simulink model "Energy_storage_blocks"  (R2025b)
settings: Solver=VariableStepAuto  StartTime=0.0  StopTime=1000  RelTol=1e-3
values from neighbouring files (symbols this model uses):
  R = 0.01    [DATA_LI_ION_CELL.mat]
undefined symbols (not defined in the file or in its folder): BATTERY_1, DC_CAPACITIVE_FILTER_1, DC_INDUCTIVE_FILTER_1, DCDC_CONVERTER_1, DCDC_CONVERTER_CONTROLLER_1, F, L
libraries: simulink x2
settings Model: Creator=barra  LastModifiedBy=DNI 76350607

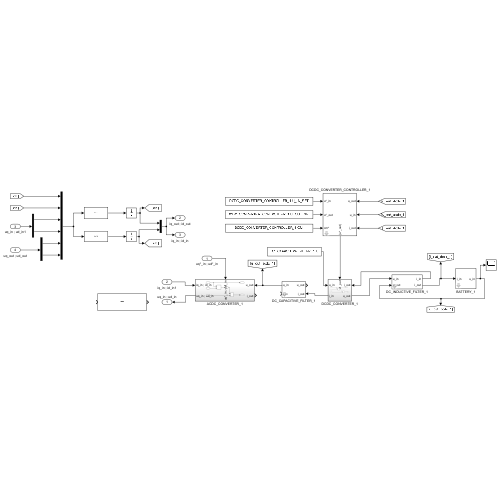
[thumbnail: Simulink's stored preview of the top-level diagram]
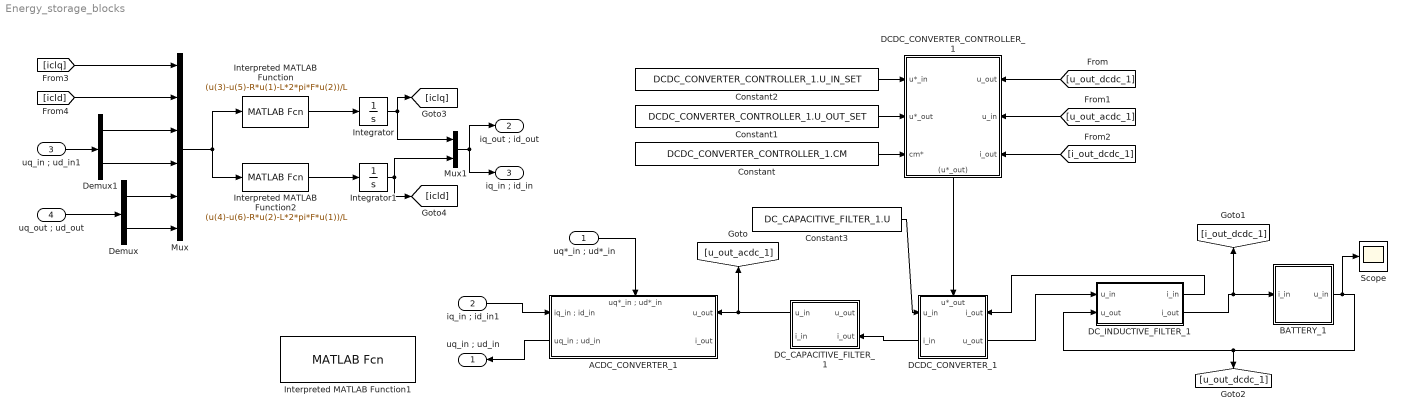
== system Energy_storage_blocks ==
  uq*_in ; ud*_in : Inport
  iq_in ; id_in1 : Inport  Port=2
  uq_in ; ud_in1 : Inport  Port=3
  uq_out ; ud_out : Inport  Port=4
  ACDC_CONVERTER_1 : Subsystem
      settings: PortSchema="{\"entries\":[{\"content\":{\"sides\":[{\"content\":{\"connectorIds\":[\"In1\",\"Out2\"]},\"type\":\"ConnectorPlacement.EquallySpacedRectSide\",\"uuid\":\"8c383f18-b1b8-414a-9022-83b924be4ee1\"},{\"content\":{\"connectorIds\":[\"In3\",\"Out1\"],\"side\":\"RIGHT\"},\"type\":\"ConnectorPlacement.EquallySpacedRectSide\",\"uuid\":\"b6aa94b4-5558-4a55-88af-197c4f32b9d6\"},{\"content\":{\"connectorIds\":[\"In2\"],\"side\":\"TOP\"},\"type\":\"ConnectorPlacement.EquallySpacedRectSide\",\"uuid\":\"f27b2a4b-2b11-4cc8-a3ae-660875af7a27\"}]},\"type\":\"ConnectorPlacement.EquallySpacedConnector\",\"uuid\":\"ed3a75f0-3b30-4418-b841-97d400508208\"}],\"packageUris\":[\"http://schema.mathworks.com/mf0/Connector/R2020b\"],\"version\":\"1.0\"}"
  BATTERY_1 : Subsystem  mask{R=BATTERY_1.R, EFF=BATTERY_1.EFF, C=BATTERY_1.C, OCV_LUT=BATTERY_1.OCV_LUT, SOC_LUT=BATTERY_1.SOC_LUT, SOC_INI=BATTERY_1.SOC_INI}
      mask prompts: R "Internal resistance (Ohm)"; EFF "Efficiency (p.u.)"; C "Capacity (Ah)"; OCV_LUT "Open Circuit Voltage OCV (V)"; SOC_LUT "Open Circuit Voltage SOC (p.u.)"; SOC_INI "Initial SOC (p.u.)"
      mask DialogControl DescTextVar Prompt: Battery.
  Constant : Constant  Value=DCDC_CONVERTER_CONTROLLER_1.CM
  Constant1 : Constant  Value=DCDC_CONVERTER_CONTROLLER_1.U_OUT_SET
  Constant2 : Constant  Value=DCDC_CONVERTER_CONTROLLER_1.U_IN_SET
  Constant3 : Constant  Value=DC_CAPACITIVE_FILTER_1.U
  DCDC_CONVERTER_1 : Subsystem
      settings: PortSchema="{\"entries\":[{\"content\":{\"sides\":[{\"content\":{\"connectorIds\":[\"In1\",\"Out2\"]},\"type\":\"ConnectorPlacement.EquallySpacedRectSide\",\"uuid\":\"16b79129-35bd-40e4-9150-a907a2dc894e\"},{\"content\":{\"connectorIds\":[\"In3\",\"Out1\"],\"side\":\"RIGHT\"},\"type\":\"ConnectorPlacement.EquallySpacedRectSide\",\"uuid\":\"aebd2ac3-6df7-4285-ab4e-40db8a096b32\"},{\"content\":{\"connectorIds\":[\"In2\"],\"side\":\"TOP\"},\"type\":\"ConnectorPlacement.EquallySpacedRectSide\",\"uuid\":\"705a8761-481f-43da-b8bb-0b2cee8f59be\"}]},\"type\":\"ConnectorPlacement.EquallySpacedConnector\",\"uuid\":\"5da3bf74-39a7-4819-a145-9938271c38b8\"}],\"packageUris\":[\"http://schema.mathworks.com/mf0/Connector/R2020b\"],\"version\":\"1.0\"}"
  DCDC_CONVERTER_CONTROLLER_1 : Subsystem  mask{I_MAX=DCDC_CONVERTER_1.I_OUT, U_IN=DCDC_CONVERTER_1.U_IN, KPU=DCDC_CONVERTER_CONTROLLER_1.KPU, KIU=DCDC_CONVERTER_CONTROLLER_1.KIU, KPI=DCDC_CONVERTER_CONTROLLER_1.KPI, KII=DCDC_CONVERTER_CONTROLLER_1.KII, INT_INI=DCDC_CONVERTER_CONTROLLER_1.INT_INI}
      mask prompts: I_MAX "Rated output current, (A)"; U_IN "Rated input voltage, (V)"; KPU "Output voltage controller, Kp (-)"; KIU "Output voltage controller, Ki (-)"; KPI "Output current controller, Kp (-)"; KII "Output current controller, Ki (-)"; INT_INI "Initial condition, current controller"
      settings: PortSchema="{\"entries\":[{\"content\":{\"sides\":[{\"content\":{\"connectorIds\":[\"In1\",\"In2\",\"In3\"]},\"type\":\"ConnectorPlacement.EquallySpacedRectSide\",\"uuid\":\"a907ae50-daf0-48ac-8972-584c22ec23bc\"},{\"content\":{\"connectorIds\":[\"In4\",\"In5\",\"In6\"],\"side\":\"RIGHT\"},\"type\":\"ConnectorPlacement.EquallySpacedRectSide\",\"uuid\":\"c451cec1-46fa-46e7-84b6-32aef918d9a7\"},{\"content\":{\"side\":\"TOP\"},\"type\":\"ConnectorPlacement.EquallySpacedRectSide\",\"uuid\":\"5fac8104-b6a5-4db9-beed-e5f35f7b50c1\"},{\"content\":{\"connectorIds\":[\"Out1\"],\"side\":\"BOTTOM\"},\"type\":\"ConnectorPlacement.EquallySpacedRectSide\",\"uuid\":\"880ffd14-00d8-4352-9ce0-8d5bb61b95c0\"}]},\"type\":\"ConnectorPlacement.EquallySpacedConnector\",\"uuid\":\"6bb2e475-6dd4-45a2-84d8-2ce6e01c7f10\"}],\"packageUris\":[\"http://schema.mathworks.com/mf0/Connector/R2020b\"],\"version\":\"1.0\"}"
      mask DialogControl DescGroupVar Prompt: Bidirectional buck-boost DCDC converter controller.
      mask DialogControl Container2 Prompt: Parameters
  DC_CAPACITIVE_FILTER_1 : Subsystem  mask{C=DC_CAPACITIVE_FILTER_1.C, U=DC_CAPACITIVE_FILTER_1.U}
      mask prompts: C "Capacitance (F)"; U "Initial voltage (V)"
      settings: PortSchema="{\"entries\":[{\"content\":{\"sides\":[{\"content\":{\"connectorIds\":[\"Out2\",\"In1\"]},\"type\":\"ConnectorPlacement.EquallySpacedRectSide\",\"uuid\":\"bcba4002-f43e-4ceb-8615-0b17579625fa\"},{\"content\":{\"connectorIds\":[\"Out1\",\"In2\"],\"side\":\"RIGHT\"},\"type\":\"ConnectorPlacement.EquallySpacedRectSide\",\"uuid\":\"6d888d39-6fd7-425a-a11e-fe4702aa9d62\"},{\"content\":{\"side\":\"TOP\"},\"type\":\"ConnectorPlacement.EquallySpacedRectSide\",\"uuid\":\"f7aa08bb-58ae-4915-b02f-c1bef0b1235c\"}]},\"type\":\"ConnectorPlacement.EquallySpacedConnector\",\"uuid\":\"fb6703e1-98b4-4d7d-a745-8e02b5eae5ed\"}],\"packageUris\":[\"http://schema.mathworks.com/mf0/Connector/R2020b\"],\"version\":\"1.0\"}"
      mask DialogControl DescGroupVar Prompt: DC capacitive filter
  DC_INDUCTIVE_FILTER_1 : Subsystem  mask{L=DC_INDUCTIVE_FILTER_1.L}
      mask prompts: L "Inductance (H)"
      mask DialogControl DescGroupVar Prompt: DC inductive filter
  Demux : Demux  Outputs=2
  Demux1 : Demux  Outputs=2
  Integrator : Integrator
  Integrator1 : Integrator
  Interpreted MATLAB Function : MATLABFcn  MATLABFcn=(u(3)-u(5)-R*u(1)-L*2*pi*F*u(2))/L  OutputDimensions=1
  Interpreted MATLAB Function1 : MATLABFcn
  Interpreted MATLAB Function2 : MATLABFcn  MATLABFcn=(u(4)-u(6)-R*u(2)-L*2*pi*F*u(1))/L  OutputDimensions=1
  Mux : Mux  Inputs=6
  Mux1 : Mux  Inputs=2
  Scope : Scope
      settings: ActiveDisplayYMinimum=577.2389529667704  ActiveDisplayYMaximum=641.19342329906692
  uq_in ; ud_in : Outport
  iq_out ; id_out : Outport  Port=2
  iq_in ; id_in : Outport  Port=3
  wires:
  BATTERY_1/1(u_in) -> Scope/1, DC_INDUCTIVE_FILTER_1/2(u_out), [u_out_dcdc_1]
  DC_INDUCTIVE_FILTER_1/2(i_out) -> [i_out_dcdc_1], BATTERY_1/1(i_in)
  DC_INDUCTIVE_FILTER_1/1(i_in) -> DCDC_CONVERTER_1/3(i_out)
  DCDC_CONVERTER_1/1(u_out) -> DC_INDUCTIVE_FILTER_1/1(u_in)
  DCDC_CONVERTER_1/2(i_in) -> DC_CAPACITIVE_FILTER_1/2(i_out)
  iq_in ; id_in1/1 -> ACDC_CONVERTER_1/1(iq_in ; id_in)
  ACDC_CONVERTER_1/2(uq_in ; ud_in) -> uq_in ; ud_in/1
  uq*_in ; ud*_in/1 -> ACDC_CONVERTER_1/2(uq*_in ; ud*_in)
  DCDC_CONVERTER_CONTROLLER_1/1((u*_out)) -> DCDC_CONVERTER_1/2(u*_out)
  [i_out_dcdc_1] -> DCDC_CONVERTER_CONTROLLER_1/6(i_out)
  [u_out_dcdc_1] -> DCDC_CONVERTER_CONTROLLER_1/4(u_out)
  Constant2/1 -> DCDC_CONVERTER_CONTROLLER_1/1(u*_in)
  Constant1/1 -> DCDC_CONVERTER_CONTROLLER_1/2(u*_out)
  Constant/1 -> DCDC_CONVERTER_CONTROLLER_1/3(cm*)
  DC_CAPACITIVE_FILTER_1/2(u_in) -> [u_out_acdc_1], ACDC_CONVERTER_1/3(u_out)
  Constant3/1 -> DCDC_CONVERTER_1/1(u_in)
  [u_out_acdc_1] -> DCDC_CONVERTER_CONTROLLER_1/5(u_in)
  Demux/2 -> Mux/6
  Demux/1 -> Mux/5
  Demux1/1 -> Mux/3
  Demux1/2 -> Mux/4
  uq_in ; ud_in1/1 -> Demux1/1
  uq_out ; ud_out/1 -> Demux/1
  Mux/1 -> Interpreted MATLAB Function/1, Interpreted MATLAB Function2/1
  Interpreted MATLAB Function/1 -> Integrator/1
  Interpreted MATLAB Function2/1 -> Integrator1/1
  Integrator1/1 -> [icld], Mux1/2
  Integrator/1 -> [iclq], Mux1/1
  Mux1/1 -> iq_in ; id_in/1, iq_out ; id_out/1
  [iclq] -> Mux/1
  [icld] -> Mux/2

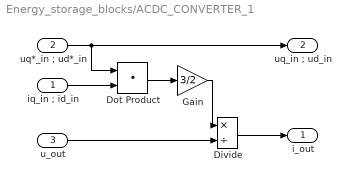
== system Energy_storage_blocks/ACDC_CONVERTER_1 ==
  iq_in ; id_in : Inport
  uq*_in ; ud*_in : Inport  Port=2
  u_out : Inport  Port=3
  Divide : Product  Inputs=*/
  Dot Product : DotProduct  OutDataTypeStr=Inherit: Inherit via internal rule
  Gain : Gain  Gain=3/2
  i_out : Outport
  uq_in ; ud_in : Outport  Port=2
  wires:
  Dot Product/1 -> Gain/1
  Gain/1 -> Divide/1
  uq*_in ; ud*_in/1 -> uq_in ; ud_in/1, Dot Product/1
  Divide/1 -> i_out/1
  u_out/1 -> Divide/2
  iq_in ; id_in/1 -> Dot Product/2

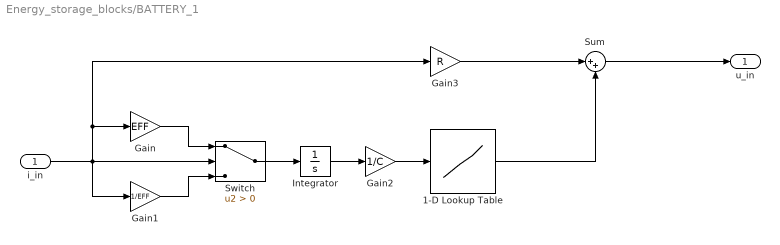
== system Energy_storage_blocks/BATTERY_1 ==
  i_in : Inport
  1-D Lookup Table : Lookup_n-D  NumberOfTableDimensions=1  BreakpointsForDimension1=SOC_LUT  Table=OCV_LUT  InternalRulePriority=Speed  RndMeth=Simplest
  Gain : Gain  Gain=EFF
  Gain1 : Gain  Gain=1/EFF
  Gain2 : Gain  Gain=1/C
  Gain3 : Gain  Gain=R
  Integrator : Integrator  InitialCondition=SOC_INI*C
  Sum : Sum  Inputs=|++
  Switch : Switch  Criteria=u2 > Threshold  SaturateOnIntegerOverflow=off  InputSameDT=off
  u_in : Outport
  wires:
  i_in/1 -> Gain1/1, Gain3/1, Gain/1, Switch/2
  Sum/1 -> u_in/1
  Gain2/1 -> 1-D Lookup Table/1
  Gain1/1 -> Switch/3
  Gain/1 -> Switch/1
  1-D Lookup Table/1 -> Sum/2
  Switch/1 -> Integrator/1
  Gain3/1 -> Sum/1
  Integrator/1 -> Gain2/1

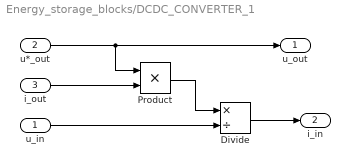
== system Energy_storage_blocks/DCDC_CONVERTER_1 ==
  u_in : Inport
  u*_out : Inport  Port=2
  i_out : Inport  Port=3
  Divide : Product  Inputs=*/
  Product : Product
  u_out : Outport
  i_in : Outport  Port=2
  wires:
  Divide/1 -> i_in/1
  Product/1 -> Divide/1
  u_in/1 -> Divide/2
  u*_out/1 -> u_out/1, Product/1
  i_out/1 -> Product/2

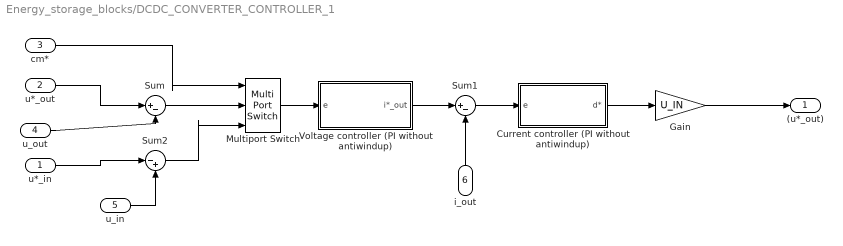
== system Energy_storage_blocks/DCDC_CONVERTER_CONTROLLER_1 ==
  u*_in : Inport
  u*_out : Inport  Port=2
  cm* : Inport  Port=3
  u_out : Inport  Port=4
  u_in : Inport  Port=5
  i_out : Inport  Port=6
  Current controller (PI without antiwindup) : Subsystem
  Gain : Gain  Gain=U_IN
  Multiport Switch : MultiPortSwitch  Inputs=2  SaturateOnIntegerOverflow=off  InputSameDT=off
  Sum : Sum  Inputs=|+-
  Sum1 : Sum  Inputs=|+-
  Sum2 : Sum  Inputs=|-+
  Voltage controller (PI without antiwindup) : Subsystem
  (u*_out) : Outport
  wires:
  Current controller (PI without antiwindup)/1(d*) -> Gain/1
  Sum/1 -> Multiport Switch/2
  i_out/1 -> Sum1/2
  Voltage controller (PI without antiwindup)/1(i*_out) -> Sum1/1
  cm*/1 -> Multiport Switch/1
  Gain/1 -> (u*_out)/1
  u_in/1 -> Sum2/2
  Sum1/1 -> Current controller (PI without antiwindup)/1(e)
  u*_out/1 -> Sum/1
  u*_in/1 -> Sum2/1
  u_out/1 -> Sum/2
  Multiport Switch/1 -> Voltage controller (PI without antiwindup)/1(e)
  Sum2/1 -> Multiport Switch/3

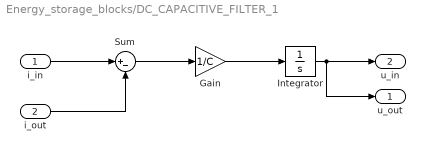
== system Energy_storage_blocks/DC_CAPACITIVE_FILTER_1 ==
  i_in : Inport
  i_out : Inport  Port=2
  Gain : Gain  Gain=1/C
  Integrator : Integrator
  Sum : Sum  Inputs=|+-
  u_out : Outport
  u_in : Outport  Port=2
  wires:
  Sum/1 -> Gain/1
  Integrator/1 -> u_out/1, u_in/1
  i_out/1 -> Sum/2
  i_in/1 -> Sum/1
  Gain/1 -> Integrator/1

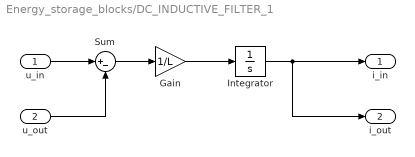
== system Energy_storage_blocks/DC_INDUCTIVE_FILTER_1 ==
  u_in : Inport
  u_out : Inport  Port=2
  Gain : Gain  Gain=1/L
  Integrator : Integrator
  Sum : Sum  Inputs=|+-
  i_in : Outport
  i_out : Outport  Port=2
  wires:
  u_out/1 -> Sum/2
  u_in/1 -> Sum/1
  Sum/1 -> Gain/1
  Integrator/1 -> i_out/1, i_in/1
  Gain/1 -> Integrator/1

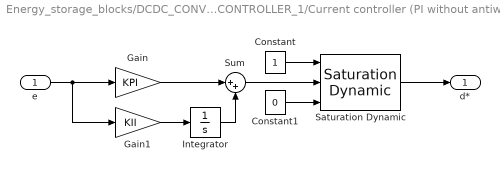
== system Energy_storage_blocks/DCDC_CONVERTER_CONTROLLER_1/Current controller (PI without antiwindup) ==
  e : Inport
  Constant : Constant
  Constant1 : Constant  Value=0
  Gain : Gain  Gain=KPI
  Gain1 : Gain  Gain=KII
  Integrator : Integrator  InitialCondition=INT_INI
  Saturation Dynamic : simulink/Discontinuities/Saturation Dynamic  OutMin=[]  OutMax=[]  OutDataTypeStr=Inherit: Same as second input  OutDataType=fixdt(1, 16)  OutScaling=2^-10  DoSatur=off
  Sum : Sum  Inputs=|++
  d* : Outport
  wires:
  Integrator/1 -> Sum/2
  Constant1/1 -> Saturation Dynamic/3
  e/1 -> Gain1/1, Gain/1
  Sum/1 -> Saturation Dynamic/2
  Gain/1 -> Sum/1
  Constant/1 -> Saturation Dynamic/1
  Gain1/1 -> Integrator/1
  Saturation Dynamic/1 -> d*/1

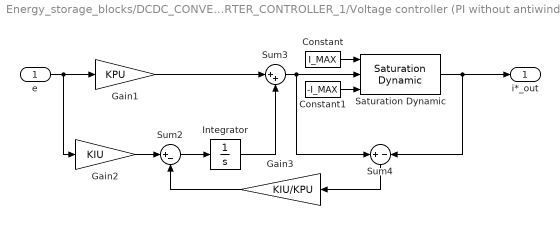
== system Energy_storage_blocks/DCDC_CONVERTER_CONTROLLER_1/Voltage controller (PI without antiwindup) ==
  e : Inport
  Constant : Constant  Value=I_MAX
  Constant1 : Constant  Value=-I_MAX
  Gain1 : Gain  Gain=KPU
  Gain2 : Gain  Gain=KIU
  Gain3 : Gain  Gain=KIU/KPU
  Integrator : Integrator
  Saturation Dynamic : simulink/Discontinuities/Saturation Dynamic  OutMin=[]  OutMax=[]  OutDataTypeStr=Inherit: Same as second input  OutDataType=fixdt(1, 16)  OutScaling=2^-10  DoSatur=off
  Sum2 : Sum  Inputs=|+-
  Sum3 : Sum  Inputs=|++
  Sum4 : Sum  Inputs=+|-
  i*_out : Outport
  wires:
  Gain1/1 -> Sum3/1
  Sum2/1 -> Integrator/1
  Integrator/1 -> Sum3/2
  Saturation Dynamic/1 -> i*_out/1, Sum4/2
  Sum3/1 -> Sum4/1, Saturation Dynamic/2
  Sum4/1 -> Gain3/1
  e/1 -> Gain2/1, Gain1/1
  Constant1/1 -> Saturation Dynamic/3
  Gain3/1 -> Sum2/2
  Constant/1 -> Saturation Dynamic/1
  Gain2/1 -> Sum2/1
